simulink model "mod_18"  (R2025a)
settings: Solver=ode45  StartTime=0.0  StopTime=15  MaxStep=1e-1  RelTol=1e-3
libraries: cstblocks x3
settings Model: Creator=fabri  LastModifiedBy=fabri

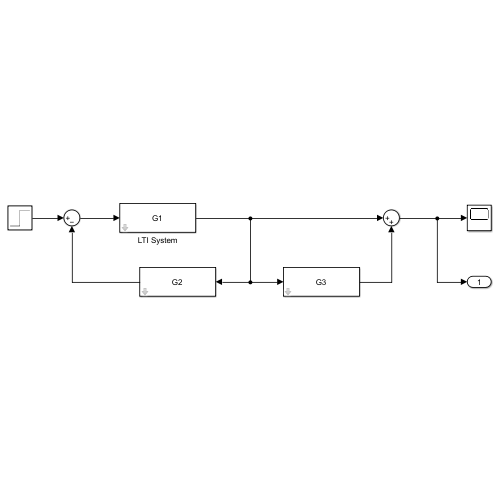
[thumbnail: Simulink's stored preview of the top-level diagram]
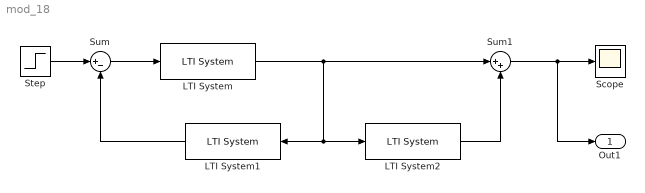
== system mod_18 ==
  LTI System : cstblocks/LTI System  sys=G1  IC=[]  PadeOrder=0
  LTI System1 : cstblocks/LTI System  sys=G2  IC=[]  PadeOrder=0
  LTI System2 : cstblocks/LTI System  sys=G3  IC=[]  PadeOrder=0
  Scope : Scope
      settings: ActiveDisplayYMinimum=-1.3392647340566697  ActiveDisplayYMaximum=2.9119176718182223
  Step : Step  Time=0  SampleTime=0
  Sum : Sum  Inputs=|+-
  Sum1 : Sum  Inputs=|++
  Out1 : Outport
  wires:
  Step/1 -> Sum/1
  Sum/1 -> LTI System/1
  LTI System1/1 -> Sum/2
  LTI System2/1 -> Sum1/2
  Sum1/1 -> Out1/1, Scope/1
  LTI System/1 -> LTI System2/1, LTI System1/1, Sum1/1
